simulink model "ball_impact"  (Simulink 8.1)
settings: Solver=ode4  SolverMode=SingleTasking  StartTime=0.0  StopTime=inf  FixedStep=0.0005  RelTol=1e-3
StartFcn:
  |  warndlg('Dexterit-E models cannot run under simulation. Please compile your model and run it from within Dexterit-E.');set_param(bdroot,'SimulationCommand','stop')
undefined symbols (not defined in the file or in its folder): CreateParameterTableGUI, slselsubs
libraries: xpclib x30, simulink x8, KINARM_general x3, KINARM_loads x2, Video x2, KINARM_EP_loads x1
(part 2 of 5)

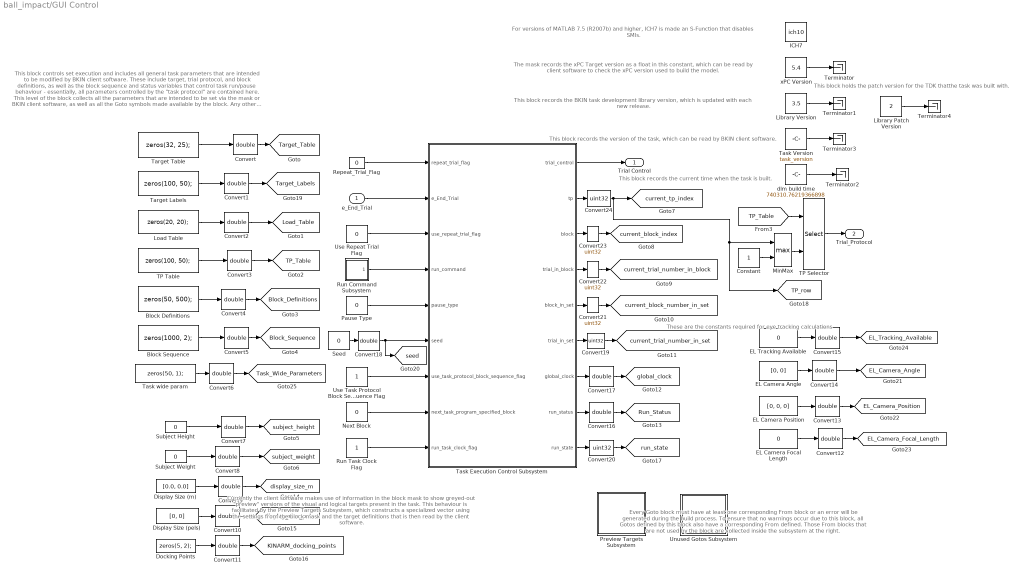
== system ball_impact/GUI Control ==
  note: This block holds the patch version for
      | the TDK thatthe task was built with.
  note: These are the constants required for eye tracking calculations
  note: This block records the version of the task,
      | which can be read by BKIN client software.
  note: This block records the BKIN task development library
      | version, which is updated with each new release.
  note: Currently the client software makes use of information in the block mask to show
      | greyed-out "preview" versions of the visual and logical targets present in the task.
      | This behaviour is facilitated by the Preview Targets Subsystem, which constructs
      | a specialized vector using the settings from the block mask and the target
      | definitions that is then read by the client software.
  note: This block controls set execution and includes all general task parameters that are intended to be modified by BKIN client software. These include
      | target, trial protocol, and block definitions, as well as the block sequence and status variables that control task run/pause behaviour - essentially, all
      | parameters controlled by the "task protocol" are contained here.
      |
      | This level of the block collects all the parameters that are intended to be set via the mask or BKIN client software, as well as all the Goto symbols
      | made available by the block. Any other parameters to be read or written outside of this block should be placed at this level. The task execution
      | control subsystem performs the actual control of task execution using these parameters.
      |
      | Those parameters used to create Goto symbols directly are collected at the left, and all other parameters are connected directly to the subsystem.
  note: The mask records the xPC Target version as a float
      | in this constant, which can be read by client software
      | to check the xPC version used to build the model.
  note: For versions of MATLAB 7.5 (R2007b) and higher,
      | ICH7 is made an S-Function that disables SMIs.
  note: Every Goto block must have at least one corresponding
      | From block or an error will be generated during the build
      | process. To ensure that no warnings occur due to this block,
      | all Gotos defined by this block also have a corresponding
      | From defined. Those From blocks that are not used by the
      | block are collected inside the subsystem at the right.
  note: This block records the current
      | time when the task is built.
  e_End_Trial : Inport
  Block Definitions : Constant  Value=zeros(50, 500);
  Block Sequence : Constant  Value=zeros(1000, 2);
  Constant : Constant  VectorParams1D=off  OutDataTypeStr=double
  Convert{,1..18} (19 alike) : DataTypeConversion  OutDataTypeStr=double
  Convert{19..24} (6 alike) : DataTypeConversion  OutDataTypeStr=uint32
  Display Size (m) : Constant  Value=[0.0, 0.0]  VectorParams1D=off  OutDataTypeStr=double
  Display Size (pels) : Constant  Value=[0, 0]  VectorParams1D=off  OutDataTypeStr=double
  Docking Points : Constant  Value=zeros(5, 2);  VectorParams1D=off  OutDataTypeStr=double
  EL Camera Angle : Constant  Value=[0, 0]  VectorParams1D=off  OutDataTypeStr=double
  EL Camera Focal Length : Constant  Value=0  VectorParams1D=off  OutDataTypeStr=double
  EL Camera Position : Constant  Value=[0, 0, 0]  VectorParams1D=off  OutDataTypeStr=double
  EL Tracking Available : Constant  Value=0  VectorParams1D=off  OutDataTypeStr=double
  ICH7 : S-Function  FunctionName=ich10  EnableBusSupport=off
  Library Patch Version : Constant  Value=2
  Library Version : Constant  Value=3.5
  Load Table : Constant  Value=zeros(20, 20);
  MinMax : MinMax  Function=max  Inputs=2
  Next Block : Constant  Value=0  VectorParams1D=off  OutDataTypeStr=double
  Pause Type : Constant  Value=0
  Preview Targets Subsystem : Subsystem
  Repeat_Trial_Flag : Constant  Value=0
  Run Command Subsystem : Subsystem
  Run Task Clock Flag : Constant  VectorParams1D=off  OutDataTypeStr=double
  Seed : Constant  Value=0
  Subject Height : Constant  Value=0  VectorParams1D=off  OutDataTypeStr=double
  Subject Weight : Constant  Value=0  VectorParams1D=off  OutDataTypeStr=double
  TP Selector : Selector  NumberOfDimensions=2  InputPortWidth=3  IndexOptions=Index vector (port),Select all  Indices=1,-1  OutputSizes=slselsubs([(-2),(-2)],1),slselsubs([(-2),(-2)],2)
  TP Table : Constant  Value=zeros(100, 50);
  Target Labels : Constant  Value=zeros(100, 50);
  Target Table : Constant  Value=zeros(32, 25);
  Task Execution Control Subsystem : Subsystem
  Task Version : Constant  Value=task_version
  Task wide param : Constant  Value=zeros(50, 1);
  Terminator{,1..4} (5 alike) : Terminator
  Unused Gotos Subsystem : Subsystem
  Use Repeat Trial Flag : Constant  Value=0
  Use Task Protocol Block Sequence Flag : Constant  VectorParams1D=off  OutDataTypeStr=double
  dlm build time : Constant  Value=740310.76219366898
  xPC Version : Constant  Value=5.4
  Trial Control : Outport
  Trial_Protocol : Outport  Port=2
  tag scope: Block_Definitions=global, Block_Sequence=global, EL_Camera_Angle=global, EL_Camera_Focal_Length=global, EL_Camera_Position=global, EL_Tracking_Available=global, KINARM_docking_points=global, Load_Table=global, Run_Status=global, TP_Table=global, TP_row=global, Target_Labels=global, Target_Table=global, Task_Wide_Parameters=global, current_block_index=global, current_block_number_in_set=global, current_tp_index=global, current_trial_number_in_block=global, current_trial_number_in_set=global, display_size_m=global, display_size_pels=global, global_clock=global, run_state=global, seed=global, subject_height=global, subject_weight=global
  wires:
  Library Patch Version/1 -> Terminator4/1
  EL Tracking Available/1 -> Convert15/1
  EL Camera Focal Length/1 -> Convert12/1
  EL Camera Position/1 -> Convert13/1
  EL Camera Angle/1 -> Convert14/1
  Task Version/1 -> Terminator3/1
  Target Labels/1 -> Convert1/1
  Task Execution Control Subsystem/9(run_state) -> Convert20/1
  Docking Points/1 -> Convert11/1
  Display Size (pels)/1 -> Convert10/1
  Display Size (m)/1 -> Convert9/1
  Constant/1 -> MinMax/2
  MinMax/1 -> TP Selector/2
  Run Task Clock Flag/1 -> Task Execution Control Subsystem/9(run_task_clock_flag)
  Use Repeat Trial Flag/1 -> Task Execution Control Subsystem/3(use_repeat_trial_flag)
  Library Version/1 -> Terminator1/1
  Subject Weight/1 -> Convert8/1
  Subject Height/1 -> Convert7/1
  Task Execution Control Subsystem/4(trial_in_block) -> Convert22/1
  Next Block/1 -> Task Execution Control Subsystem/8(next_task_program_specified_block)
  Block Sequence/1 -> Convert5/1
  TP Table/1 -> Convert3/1
  xPC Version/1 -> Terminator/1
  Target Table/1 -> Convert/1
  Block Definitions/1 -> Convert4/1
  Task Execution Control Subsystem/5(block_in_set) -> Convert21/1
  Use Task Protocol Block Sequence Flag/1 -> Task Execution Control Subsystem/7(use_task_protocol_block_sequence_flag)
  [TP_Table] -> TP Selector/1
  Task Execution Control Subsystem/6(trial_in_set) -> Convert19/1
  Task Execution Control Subsystem/3(block) -> Convert23/1
  Pause Type/1 -> Task Execution Control Subsystem/5(pause_type)
  Run Command Subsystem/1(Out1) -> Task Execution Control Subsystem/4(run_command)
  Seed/1 -> Convert18/1
  e_End_Trial/1 -> Task Execution Control Subsystem/2(e_End_Trial)
  TP Selector/1 -> Trial_Protocol/1
  Task Execution Control Subsystem/2(tp) -> Convert24/1
  Task Execution Control Subsystem/1(trial_control) -> Trial Control/1
  Load Table/1 -> Convert2/1
  Task Execution Control Subsystem/7(global_clock) -> Convert17/1
  Task Execution Control Subsystem/8(run_status) -> Convert16/1
  dlm build time/1 -> Terminator2/1
  Task wide param/1 -> Convert6/1
  Convert/1 -> [Target_Table]
  Convert1/1 -> [Target_Labels]
  Convert2/1 -> [Load_Table]
  Convert3/1 -> [TP_Table]
  Convert4/1 -> [Block_Definitions]
  Convert5/1 -> [Block_Sequence]
  Convert6/1 -> [Task_Wide_Parameters]
  Convert7/1 -> [subject_height]
  Convert8/1 -> [subject_weight]
  Convert9/1 -> [display_size_m]
  Convert10/1 -> [display_size_pels]
  Convert11/1 -> [KINARM_docking_points]
  Convert12/1 -> [EL_Camera_Focal_Length]
  Convert13/1 -> [EL_Camera_Position]
  Convert14/1 -> [EL_Camera_Angle]
  Convert15/1 -> [EL_Tracking_Available]
  Convert16/1 -> [Run_Status]
  Convert17/1 -> [global_clock]
  Convert18/1 -> [seed], Task Execution Control Subsystem/6(seed)
  Convert20/1 -> [run_state]
  Convert19/1 -> [current_trial_number_in_set]
  Convert21/1 -> [current_block_number_in_set]
  Convert22/1 -> [current_trial_number_in_block]
  Convert23/1 -> [current_block_index]
  Convert24/1 -> [TP_row], MinMax/1, [current_tp_index]
  Repeat_Trial_Flag/1 -> Task Execution Control Subsystem/1(repeat_trial_flag)

== system ball_impact/Parameter Table Defn ==
  TP_table : Subsystem
  buttons : Subsystem
  events : Subsystem
  load_table : Subsystem
  target_table : Subsystem
  task_definition : Subsystem
  task_wide : Subsystem

== system ball_impact/DataLogging/Create Analog Inputs Subsystem ==
  In1 : Inport
  Analog Data : DataTypeConversion  SaturateOnIntegerOverflow=on  RndMeth=Zero
  Analog Data Width : DataTypeConversion  SaturateOnIntegerOverflow=on  RndMeth=Zero
  Mux2 : Mux  Inputs=2
  Not Logging Analog Inputs : Constant  Value=0
  Rate Transition9 : RateTransition
  Subtract : Sum  Inputs=-+
  Width : Width
  Out1 : Outport
  wires:
  Mux2/1 -> Rate Transition9/1
  In1/1 -> Analog Data/1, Width/1
  Subtract/1 -> Analog Data Width/1
  Not Logging Analog Inputs/1 -> Subtract/1
  Analog Data Width/1 -> Mux2/1
  Width/1 -> Subtract/2
  Analog Data/1 -> Mux2/2
  Rate Transition9/1 -> Out1/1

== system ball_impact/DataLogging/Create Custom Data Subsystem ==
  In1 : Inport
  Custom Data : DataTypeConversion  SaturateOnIntegerOverflow=on  RndMeth=Zero
  Custom Data Width : DataTypeConversion  SaturateOnIntegerOverflow=on  RndMeth=Zero
  Mux6 : Mux  Inputs=2
  Rate Transition9 : RateTransition
  Width : Width
  Out1 : Outport
  wires:
  Mux6/1 -> Rate Transition9/1
  In1/1 -> Custom Data/1, Width/1
  Custom Data Width/1 -> Mux6/1
  Width/1 -> Custom Data Width/1
  Custom Data/1 -> Mux6/2
  Rate Transition9/1 -> Out1/1

== system ball_impact/DataLogging/Create Event Codes Subsystem ==
  In1 : Inport
  Event Codes : DataTypeConversion  SaturateOnIntegerOverflow=on  RndMeth=Zero
  Mux4 : Mux  Inputs=2
  Not Logging Event Codes : Constant  Value=0
  Number of Event Codes : DataTypeConversion  SaturateOnIntegerOverflow=on  RndMeth=Zero
  Rate Transition9 : RateTransition
  Subtract : Sum  Inputs=-+
  Width : Width
  Out1 : Outport
  wires:
  Mux4/1 -> Rate Transition9/1
  In1/1 -> Event Codes/1, Width/1
  Not Logging Event Codes/1 -> Subtract/1
  Subtract/1 -> Number of Event Codes/1
  Width/1 -> Subtract/2
  Number of Event Codes/1 -> Mux4/1
  Event Codes/1 -> Mux4/2
  Rate Transition9/1 -> Out1/1

== system ball_impact/DataLogging/Create KINARM Data Subsystem ==
  In1 : Inport
  Arm Kinematics : DataTypeConversion  SaturateOnIntegerOverflow=on  RndMeth=Zero
  Kinarm Data Width : DataTypeConversion  SaturateOnIntegerOverflow=on  RndMeth=Zero
  Mux : Mux  Inputs=3
  Mux1 : Mux  Inputs=2
  Mux3 : Mux
  Rate Transition4 : RateTransition
  Select Arm Data : Selector  NumberOfDimensions=2  InputPortWidth=3  IndexOptions=Index vector (dialog),Index vector (dialog)  Indices=[1, 2],[17,18,19,20,21,22,23,24,15,16, 44, 45, 46, 47, 48, 49, 50]  OutputSizes=slselsubs([(-2),(-2)],1),slselsubs([(-2),(-2)],2)
  Select Arm1 : Selector  NumberOfDimensions=2  InputPortWidth=3  IndexOptions=Index vector (dialog),Select all  Indices=1,-1  OutputSizes=slselsubs([(-2),(-2)],1),slselsubs([(-2),(-2)],2)
  Select Arm2 : Selector  NumberOfDimensions=2  InputPortWidth=3  IndexOptions=Index vector (dialog),Select all  Indices=2,-1  OutputSizes=slselsubs([(-2),(-2)],1),slselsubs([(-2),(-2)],2)
  Width : Width
  Out1 : Outport
  wires:
  Select Arm Data/1 -> Select Arm2/1, Select Arm1/1
  In1/1 -> Select Arm Data/1
  Mux1/1 -> Rate Transition4/1
  Mux3/1 -> Width/1, Arm Kinematics/1
  Select Arm2/1 -> Mux3/2
  Select Arm1/1 -> Mux3/1
  Kinarm Data Width/1 -> Mux1/1
  Width/1 -> Kinarm Data Width/1
  Arm Kinematics/1 -> Mux1/2
  [ForcePlateData] -> Mux3/4
  [Gaze_Global] -> Mux/1
  Mux/1 -> Mux3/3
  [Gaze_Event_Info] -> Mux/3
  [Gaze_pupil_area] -> Mux/2
  Rate Transition4/1 -> Out1/1

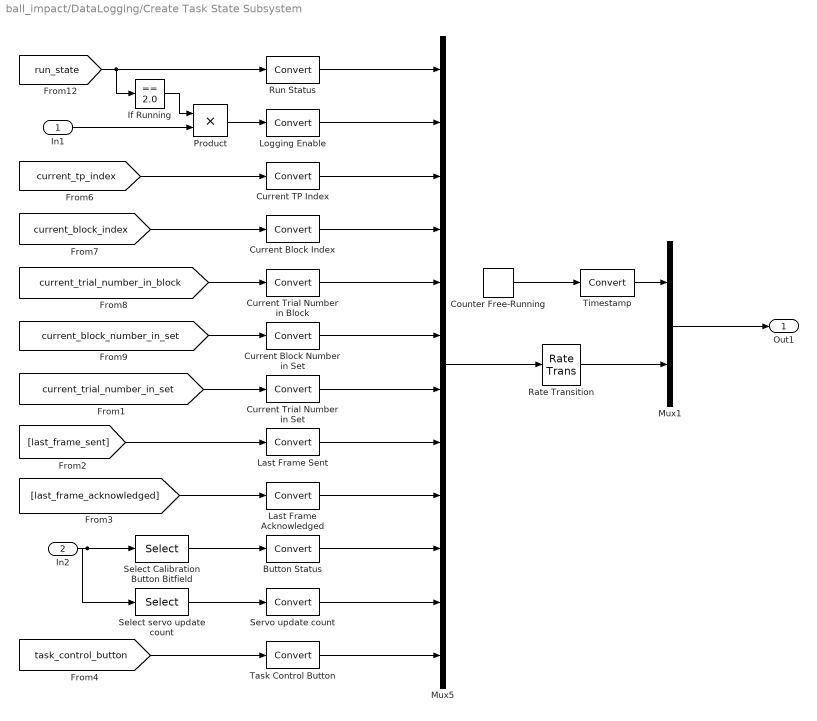
== system ball_impact/DataLogging/Create Task State Subsystem ==
  In1 : Inport
  In2 : Inport  Port=2
  Button Status : DataTypeConversion  SaturateOnIntegerOverflow=on  RndMeth=Zero
  Counter Free-Running : simulink/Sources/Counter Free-Running  NumBits=32  tsamp=-1
  Current Block Index : DataTypeConversion  SaturateOnIntegerOverflow=on  RndMeth=Zero
  Current Block Number in Set : DataTypeConversion  SaturateOnIntegerOverflow=on  RndMeth=Zero
  Current TP Index : DataTypeConversion  SaturateOnIntegerOverflow=on  RndMeth=Zero
  Current Trial Number in Block : DataTypeConversion  SaturateOnIntegerOverflow=on  RndMeth=Zero
  Current Trial Number in Set : DataTypeConversion  SaturateOnIntegerOverflow=on  RndMeth=Zero
  If Running : simulink/Logic and Bit Operations/Compare To Constant  relop===  const=2.0  OutDataTypeStr=uint8  ZeroCross=off
  Last Frame Acknowledged : DataTypeConversion  SaturateOnIntegerOverflow=on  RndMeth=Zero
  Last Frame Sent : DataTypeConversion  SaturateOnIntegerOverflow=on  RndMeth=Zero
  Logging Enable : DataTypeConversion  SaturateOnIntegerOverflow=on  RndMeth=Zero
  Mux1 : Mux  Inputs=2
  Mux5 : Mux  Inputs=12
  Product : Product  RndMeth=Zero
  Rate Transition : RateTransition
  Run Status : DataTypeConversion  SaturateOnIntegerOverflow=on  RndMeth=Zero
  Select Calibration Button Bitfield : Selector  NumberOfDimensions=2  InputPortWidth=3  IndexOptions=Index vector (dialog),Index vector (dialog)  Indices=[3],[13]  OutputSizes=slselsubs([(-2),(-2)],1),slselsubs([(-2),(-2)],2)
  Select servo update count : Selector  NumberOfDimensions=2  InputPortWidth=3  IndexOptions=Index vector (dialog),Index vector (dialog)  Indices=[3],[12]  OutputSizes=slselsubs([(-2),(-2)],1),slselsubs([(-2),(-2)],2)
  Servo update count : DataTypeConversion  SaturateOnIntegerOverflow=on  RndMeth=Zero
  Task Control Button : DataTypeConversion  SaturateOnIntegerOverflow=on  RndMeth=Zero
  Timestamp : DataTypeConversion  SaturateOnIntegerOverflow=on  RndMeth=Zero
  Out1 : Outport
  wires:
  Task Control Button/1 -> Mux5/12
  [task_control_button] -> Task Control Button/1
  In2/1 -> Select Calibration Button Bitfield/1, Select servo update count/1
  Button Status/1 -> Mux5/10
  Select Calibration Button Bitfield/1 -> Button Status/1
  [last_frame_acknowledged] -> Last Frame Acknowledged/1
  [last_frame_sent] -> Last Frame Sent/1
  Last Frame Acknowledged/1 -> Mux5/9
  Last Frame Sent/1 -> Mux5/8
  In1/1 -> Product/2
  Current Trial Number in Set/1 -> Mux5/7
  Current Block Number in Set/1 -> Mux5/6
  Current Trial Number in Block/1 -> Mux5/5
  Current Block Index/1 -> Mux5/4
  Current TP Index/1 -> Mux5/3
  Logging Enable/1 -> Mux5/2
  Run Status/1 -> Mux5/1
  [current_trial_number_in_set] -> Current Trial Number in Set/1
  [current_block_number_in_set] -> Current Block Number in Set/1
  [current_trial_number_in_block] -> Current Trial Number in Block/1
  [current_block_index] -> Current Block Index/1
  [current_tp_index] -> Current TP Index/1
  If Running/1 -> Product/1
  Counter Free-Running/1 -> Timestamp/1
  [run_state] -> If Running/1, Run Status/1
  Product/1 -> Logging Enable/1
  Servo update count/1 -> Mux5/11
  Select servo update count/1 -> Servo update count/1
  Mux1/1 -> Out1/1
  Timestamp/1 -> Mux1/1
  Mux5/1 -> Rate Transition/1
  Rate Transition/1 -> Mux1/2

== system ball_impact/DataLogging/Keep alive ==
  note: Every 100ms this sends out a message that
      | DexDisplay should get and replay to Dex.
      | That is how Dex can tell if DexDisplay is blocked by a firewall.
  Pack : xpclib/UDP/Pack  datatypes={'double'}  byteAlign=1
  Send : xpclib/UDP/Send  ipAddress=192.168.0.1  ipPort=50010  localPort=-1  vblLen=off  sampletime=0.1
  const : Constant  Value=[1 1 1 1 1]  OutDataTypeStr=double
  wires:
  const/1 -> Pack/1
  Pack/1 -> Send/1

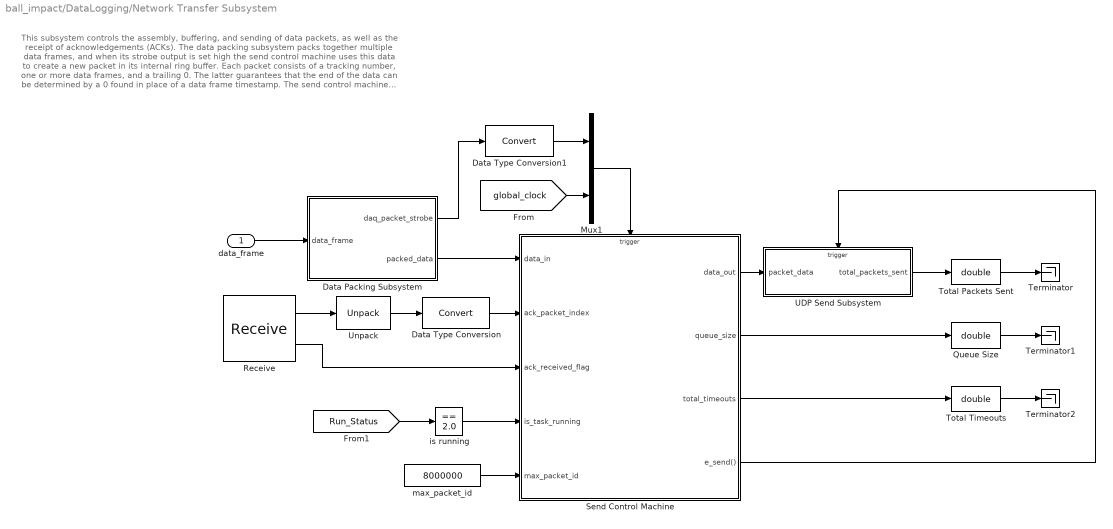
== system ball_impact/DataLogging/Network Transfer Subsystem ==
  note: This subsystem controls the assembly, buffering, and sending of data packets, as well as the receipt of acknowledgements (ACKs). The data packing subsystem packs
      | together multiple data frames, and when its strobe output is set high the send control machine uses this data to create a new packet in its internal ring buffer. Each
      | packet consists of a tracking number, one or more data frames, and a trailing 0. The latter guarantees that the end of the data can be determined by a 0 found in
      | place of a data frame timestamp.
      |
      | The send control machine will send the next packet in its buffer after an ACK for the previous one is received. If it  will resend a packet if it has not received an ACK
      | after a fixed time, and repeat the send for every elapse of that time. Currently up to 5000 packets - a minimum of 5 seconds and a maximum of 30 seconds of data,
      | depending on frame size - are buffered.
  data_frame : Inport
  Data Packing Subsystem : Subsystem  TreatAsAtomicUnit=on  SystemSampleTime=0.001
  Data Type Conversion : DataTypeConversion
  Data Type Conversion1 : DataTypeConversion
  Mux1 : Mux  Inputs=2
  Queue Size : DataTypeConversion  OutDataTypeStr=double  SaturateOnIntegerOverflow=on  RndMeth=Zero
  Receive : xpclib/UDP/Receive  ipAddress=192.168.0.1  ipPort=50001  width=4  vblLen=off  sampletime=BKIN_STEP_TIME
  Send Control Machine : Stateflow chart  TreatAsAtomicUnit=on
  Terminator : Terminator
  Terminator1 : Terminator
  Terminator2 : Terminator
  Total Packets Sent : DataTypeConversion  OutDataTypeStr=double  SaturateOnIntegerOverflow=on  RndMeth=Zero
  Total Timeouts : DataTypeConversion  OutDataTypeStr=double  SaturateOnIntegerOverflow=on  RndMeth=Zero
  UDP Send Subsystem : Subsystem  TreatAsAtomicUnit=on
  Unpack : xpclib/UDP/Unpack  dimensions={[1]}  datatypes={'single'}  byteAlign=1
  is running : simulink/Logic and Bit Operations/Compare To Constant  relop===  const=2.0  OutDataTypeStr=uint8  ZeroCross=off
  max_packet_id : Constant  Value=8000000  OutDataTypeStr=uint32
  wires:
  is running/1 -> Send Control Machine/4(is_task_running)
  [Run_Status] -> is running/1
  Data Type Conversion1/1 -> Mux1/1
  Total Packets Sent/1 -> Terminator/1
  Queue Size/1 -> Terminator1/1
  Data Type Conversion/1 -> Send Control Machine/2(ack_packet_index)
  Receive/2 -> Send Control Machine/3(ack_received_flag)
  Send Control Machine/1(data_out) -> UDP Send Subsystem/1(packet_data)
  Send Control Machine/4(e_send()) -> UDP Send Subsystem/Trigger
  Data Packing Subsystem/1(daq_packet_strobe) -> Data Type Conversion1/1
  [global_clock] -> Mux1/2
  Send Control Machine/2(queue_size) -> Queue Size/1
  Send Control Machine/3(total_timeouts) -> Total Timeouts/1
  Mux1/1 -> Send Control Machine/Trigger
  Receive/1 -> Unpack/1
  Unpack/1 -> Data Type Conversion/1
  Data Packing Subsystem/2(packed_data) -> Send Control Machine/1(data_in)
  data_frame/1 -> Data Packing Subsystem/1(data_frame)
  UDP Send Subsystem/1(total_packets_sent) -> Total Packets Sent/1
  Total Timeouts/1 -> Terminator2/1
  max_packet_id/1 -> Send Control Machine/5(max_packet_id)

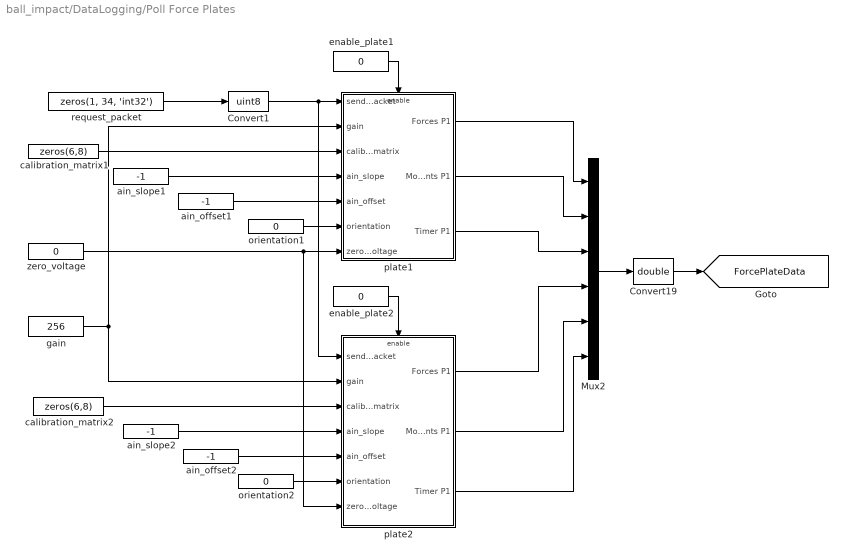
== system ball_impact/DataLogging/Poll Force Plates ==
  Convert1 : DataTypeConversion  OutDataTypeStr=uint8
  Convert19 : DataTypeConversion  OutDataTypeStr=double
  Mux2 : Mux  Inputs=6
  ain_offset1 : Constant  Value=-1
  ain_offset2 : Constant  Value=-1
  ain_slope1 : Constant  Value=-1
  ain_slope2 : Constant  Value=-1
  calibration_matrix1 : Constant  Value=zeros(6,8)
  calibration_matrix2 : Constant  Value=zeros(6,8)
  enable_plate1 : Constant  Value=0
  enable_plate2 : Constant  Value=0
  gain : Constant  Value=256
  orientation1 : Constant  Value=0
  orientation2 : Constant  Value=0
  plate1 : Subsystem
  plate2 : Subsystem
  request_packet : Constant  Value=zeros(1, 34, 'int32')
  zero_voltage : Constant  Value=0
  tag scope: ForcePlateData=global
  wires:
  gain/1 -> plate2/2(gain), plate1/2(gain)
  plate1/1(Forces P1) -> Mux2/1
  plate1/2(Moments P1) -> Mux2/2
  plate1/3(Timer P1) -> Mux2/3
  plate2/1(Forces P1) -> Mux2/4
  plate2/2(Moments P1) -> Mux2/5
  plate2/3(Timer P1) -> Mux2/6
  calibration_matrix1/1 -> plate1/3(calib_matrix)
  calibration_matrix2/1 -> plate2/3(calib_matrix)
  enable_plate1/1 -> plate1/Enable
  enable_plate2/1 -> plate2/Enable
  Mux2/1 -> Convert19/1
  ain_slope1/1 -> plate1/4(ain_slope)
  ain_offset1/1 -> plate1/5(ain_offset)
  ain_slope2/1 -> plate2/4(ain_slope)
  ain_offset2/1 -> plate2/5(ain_offset)
  orientation1/1 -> plate1/6(orientation)
  orientation2/1 -> plate2/6(orientation)
  Convert19/1 -> [ForcePlateData]
  Convert1/1 -> plate1/1(send_packet), plate2/1(send_packet)
  request_packet/1 -> Convert1/1
  zero_voltage/1 -> plate1/7(zero_voltage), plate2/7(zero_voltage)

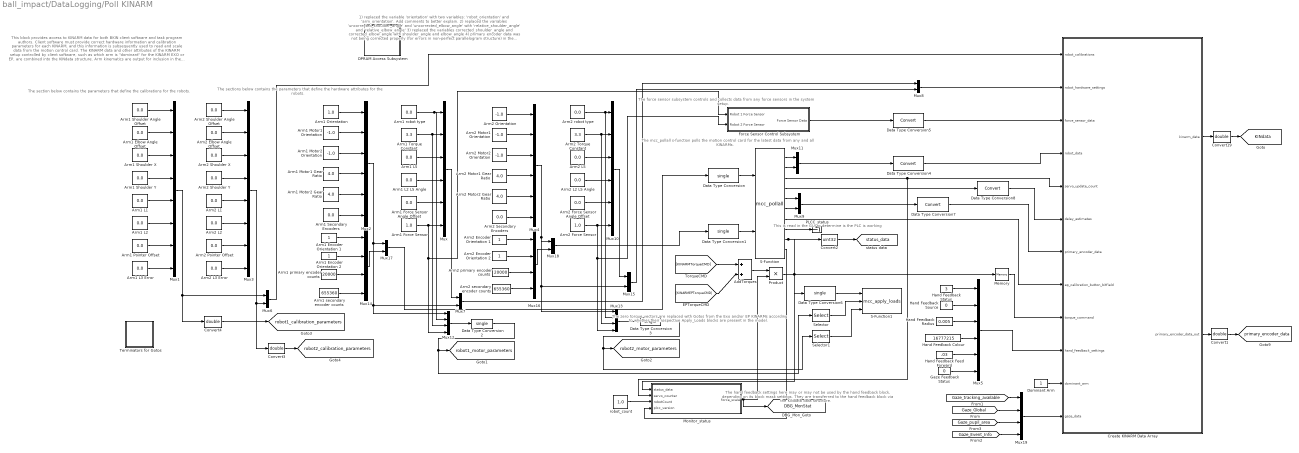
== system ball_impact/DataLogging/Poll KINARM ==
  note: This block provides access to KINARM data for both BKIN client software and task program authors. Client software must provide
      | correct hardware information and calibration parameters for each KINARM, and this information is subsequently used to read
      | and scale data from the motion control card. The KINARM data and other attributes of the KINARM setup controlled by client
      | software, such as which arm is "dominant" for the KINARM EXO or EP, are combined into the KINdata structure. Arm kinematics
      | are output for inclusion in the current data frame.
      |
      | This block also offers client software access to the motion control card DPRAM via the DPRAM access subsystem.
      |
      | Note: The mask replaces the ZeroTorque constant with a From block that includes the commanded torques providing the model
      | includes an instance of the load-applying block.
      |
      | Note: For each Goto block created here, a corresponding From block is included in the Terminators for Gotos subsystem. This is
      | solely to prevent unnecessary warnings at the Matlab prompt if such From blocks are not present.
  note: The mcc_pollall s-function polls the motion control
      | card for the latest data from any and all KINARMs.
  note: The section below contains the parameters that define the calibrations for the robots.
  note: The sections below contains the parameters that define the hardware attributes for the robots.
  note: The hand feedback settings here may or may not be used by the hand
      | feedback block, depending on its block mask settings. They are
      | transferred to the hand feedback block via the KINdata data structure.
  note: The force sensor subsystem controls and collects
      | data from any force sensors in the system setup.
  note: The zero torque vectors are replaced with Gotos
      | from the Exo and/or EP KINARMs according to
      | whether their respective Apply_Loads blocks are
      | present in the model.
  note: 1) replaced the variable 'orientation' with two variables: 'robot_orientation' and 'arm_orientation'.  Add comments to better explain.
      | 2) replaced the variables 'uncorrected_shoulder_angle' and 'uncorrected_elbow_angle' with 'relative_shoulder_angle' and 'relative_elbow_angle'
      | 3) replaced the variables corrected_shoulder_angle and corrected_elbow_angle with shoulder_angle and elbow_angle
      | 4) primary encoder data was not being corrected properly (for errors in non-perfect parallelogram structure) in the original.  This has now been fixed.
      | 5) replaced "if (robot_type < 1.0 && orientation == 2) || (robot_type > 0.0 && orientation == 1)"
      |             with "(robot_orientation == -1)"
  note: This is read in the GUI to determine is the PLC is working
  AddTorques : Sum
  Arm1 Elbow Angle Offset : Constant  Value=0.0
  Arm1 Encoder Orientation 1 : Constant
  Arm1 Encoder Orientation 2 : Constant
  Arm1 Force Sensor : Constant  Value=1.0
  Arm1 Force Sensor Angle Offset : Constant  Value=0.0
  Arm1 L1 : Constant  Value=0.0
  Arm1 L2 : Constant  Value=0.0
  Arm1 L2 L5 Angle : Constant  Value=0.0
  Arm1 L3 Error : Constant  Value=0.0
  Arm1 L5 : Constant  Value=0.0
  Arm1 Motor1 Gear Ratio : Constant  Value=4.0
  Arm1 Motor1 Orientation : Constant  Value=-1.0
  Arm1 Motor2 Gear Ratio : Constant  Value=4.0
  Arm1 Motor2 Orientation : Constant  Value=-1.0
  Arm1 Orientation : Constant  Value=1.0
  Arm1 Pointer Offset : Constant  Value=0.0
  Arm1 Secondary Encoders : Constant  Value=0.0
  Arm1 Shoulder Angle Offset : Constant  Value=0.0
  Arm1 Shoulder X : Constant  Value=0.0
  Arm1 Shoulder Y : Constant  Value=0.0
  Arm1 Torque Constant : Constant  Value=3.3
  Arm1 primary encoder counts : Constant  Value=20000
  Arm1 robot type : Constant  Value=0.0
  Arm1 secondary encoder counts : Constant  Value=655360
  Arm2 Elbow Angle Offset : Constant  Value=0.0
  Arm2 Encoder Orientation 1 : Constant
  Arm2 Encoder Orientation 2 : Constant
  Arm2 Force Sensor : Constant  Value=1.0
  Arm2 Force Sensor Angle Offset : Constant  Value=0.0
  Arm2 L1 : Constant  Value=0.0
  Arm2 L2 : Constant  Value=0.0
  Arm2 L2 L5 Angle : Constant  Value=0.0
  Arm2 L3 Error : Constant  Value=0.0
  Arm2 L5 : Constant  Value=0.0
  Arm2 Motor1 Gear Ratio : Constant  Value=4.0
  Arm2 Motor1 Orientation : Constant  Value=-1.0
  Arm2 Motor2 Gear Ratio : Constant  Value=4.0
  Arm2 Motor2 Orientation : Constant  Value=-1.0
  Arm2 Orientation : Constant  Value=-1.0
  Arm2 Pointer Offset : Constant  Value=0.0
  Arm2 Secondary Encoders : Constant  Value=0.0
  Arm2 Shoulder Angle Offset : Constant  Value=0.0
  Arm2 Shoulder X : Constant  Value=0.0
  Arm2 Shoulder Y : Constant  Value=0.0
  Arm2 Torque Constant : Constant  Value=3.3
  Arm2 primary encoder counts : Constant  Value=20000
  Arm2 robot type : Constant  Value=0.0
  Arm2 secondary encoder counts : Constant  Value=655360
  Convert{1,3..4,19} (4 alike) : DataTypeConversion  OutDataTypeStr=double
  Convert2 : DataTypeConversion  OutDataTypeStr=uint32
  Create KINARM Data Array : MATLAB Function  TreatAsAtomicUnit=on
  DPRAM Access Subsystem : Subsystem
  Data Type Conversion{,1..3,6} (5 alike) : DataTypeConversion  OutDataTypeStr=single
  Data Type Conversion{4..5,7..8} (4 alike) : DataTypeConversion
  Dominant Arm : Constant
  Force Sensor Control Subsystem : Subsystem
  Gaze Feedback Status : Constant  Value=0
  Hand Feedback Colour : Constant  Value=16777215
  Hand Feedback Feed Forward : Constant  Value=.03
  Hand Feedback Radius : Constant  Value=0.005
  Hand Feedback Source : Constant  Value=0
  Hand Feedback Status : Constant  Value=3
  Memory : Memory
  Monitor_status : MATLAB Function  TreatAsAtomicUnit=on  SystemSampleTime=.001
  Mux{,2,4..5,10} (5 alike) : Mux  Inputs=6
  Mux1 : Mux  Inputs=8
  Mux{6..9,11,15,17..18} (8 alike) : Mux  Inputs=2
  Mux{12..14,16,19} (5 alike) : Mux
  Mux3 : Mux  Inputs=8
  PLCC_status : Terminator
  Product : Product  RndMeth=Zero
  S-Function : S-Function  FunctionName=mcc_pollall  EnableBusSupport=off
  S-Function1 : S-Function  FunctionName=mcc_apply_loads  EnableBusSupport=off
  Selector : Selector  InputPortWidth=9  IndexOptions=Index vector (dialog)  Indices=[1, 2, 3, 4, 5, 8]  OutputSizes=[(-2)]
  Selector1 : Selector  InputPortWidth=9  IndexOptions=Index vector (dialog)  Indices=[1, 2, 3, 4, 5, 8]  OutputSizes=[(-2)]
  Terminators for Gotos : Subsystem
  robot_count : Constant  Value=1.0
  tag scope: DBG_MonStat=global, KINdata=global, primary_encoder_data=global, robot1_calibration_parameters=global, robot1_motor_parameters=global, robot2_calibration_parameters=global, robot2_motor_parameters=global, status_data=global
  wires:
  Arm2 secondary encoder counts/1 -> Mux16/4
  Arm2 primary encoder counts/1 -> Mux16/3
  Arm1 secondary encoder counts/1 -> Mux14/4
  Arm1 primary encoder counts/1 -> Mux14/3
  Arm1 Shoulder Angle Offset/1 -> Mux1/1
  Arm1 Elbow Angle Offset/1 -> Mux1/2
  Arm1 Shoulder X/1 -> Mux1/3
  Arm1 Shoulder Y/1 -> Mux1/4
  Arm1 L1/1 -> Mux1/5
  Arm1 L2/1 -> Mux1/6
  Arm1 Pointer Offset/1 -> Mux1/7
  Arm1 L3 Error/1 -> Mux1/8
  Arm2 Shoulder Angle Offset/1 -> Mux3/1
  Arm2 Elbow Angle Offset/1 -> Mux3/2
  Arm2 Shoulder X/1 -> Mux3/3
  Arm2 Shoulder Y/1 -> Mux3/4
  Arm2 L1/1 -> Mux3/5
  Arm2 L2/1 -> Mux3/6
  Arm2 Pointer Offset/1 -> Mux3/7
  Arm2 L3 Error/1 -> Mux3/8
  Hand Feedback Status/1 -> Mux5/1
  Hand Feedback Source/1 -> Mux5/2
  Hand Feedback Radius/1 -> Mux5/3
  Hand Feedback Colour/1 -> Mux5/4
  Hand Feedback Feed Forward/1 -> Mux5/5
  Create KINARM Data Array/1(kinarm_data) -> Convert19/1
  Arm1 Orientation/1 -> Mux2/1
  Arm1 Motor1 Orientation/1 -> Mux2/2
  Arm1 Motor2 Orientation/1 -> Mux2/3
  Arm1 Motor1 Gear Ratio/1 -> Mux2/4
  Arm1 Motor2 Gear Ratio/1 -> Mux2/5
  Arm1 Secondary Encoders/1 -> Mux2/6
  Arm2 Orientation/1 -> Mux4/1
  Arm2 Motor1 Orientation/1 -> Mux4/2
  Arm2 Motor2 Orientation/1 -> Mux4/3
  Arm2 Motor1 Gear Ratio/1 -> Mux4/4
  Arm2 Motor2 Gear Ratio/1 -> Mux4/5
  Arm2 Secondary Encoders/1 -> Mux4/6
  Arm1 robot type/1 -> Mux/1, Mux12/2
  Arm1 Torque Constant/1 -> Mux/2, Mux12/3
  Arm1 L5/1 -> Mux/3
  Arm1 L2 L5 Angle/1 -> Mux/4
  Arm2 robot type/1 -> Mux10/1, Mux13/2
  Arm2 Torque Constant/1 -> Mux10/2, Mux13/3
  Arm2 L5/1 -> Mux10/3
  Arm2 L2 L5 Angle/1 -> Mux10/4
  Arm2 Force Sensor/1 -> Mux10/6, Force Sensor Control Subsystem/2(Robot 2 Force Sensor), Mux13/4
  Dominant Arm/1 -> Create KINARM Data Array/11(dominant_arm)
  Memory/1 -> Create KINARM Data Array/9(torque_command)
  Mux5/1 -> Create KINARM Data Array/10(hand_feedback_settings)
  Mux/1 -> Mux7/1
  Mux2/1 -> Mux17/1, Mux12/1, Mux7/2
  Mux10/1 -> Mux15/1
  Mux4/1 -> Mux18/1, Mux13/1, Mux15/2
  Mux11/1 -> Data Type Conversion4/1
  Force Sensor Control Subsystem/1(Force Sensor Data) -> Data Type Conversion5/1
  Arm1 Force Sensor/1 -> Mux/6, Force Sensor Control Subsystem/1(Robot 1 Force Sensor), Mux12/4
  Arm1 Force Sensor Angle Offset/1 -> Mux/5
  Arm2 Force Sensor Angle Offset/1 -> Mux10/5
  Mux7/1 -> Mux8/1
  Mux15/1 -> Mux8/2
  Mux8/1 -> Create KINARM Data Array/2(robot_hardware_settings)
  S-Function/1 -> Mux11/1
  S-Function/2 -> Mux11/2
  S-Function/3 -> Create KINARM Data Array/5(servo_update_count), Monitor_status/2(servo_counter)
  S-Function/4 -> Data Type Conversion8/1
  Data Type Conversion1/1 -> S-Function/2
  Mux9/1 -> Data Type Conversion7/1
  Mux1/1 -> Mux6/1, Convert4/1
  Mux3/1 -> Mux6/2, Convert3/1
  Mux6/1 -> Create KINARM Data Array/1(robot_calibrations)
  Data Type Conversion/1 -> S-Function/1
  Mux12/1 -> Data Type Conversion2/1
  Data Type Conversion2/1 -> [robot1_motor_parameters], Selector/1
  Mux13/1 -> Data Type Conversion3/1
  Data Type Conversion3/1 -> [robot2_motor_parameters], Selector1/1
  S-Function/5 -> Mux9/1
  S-Function/6 -> Mux9/2
  S-Function/7 -> Create KINARM Data Array/8(ep_calibration_button_bitfield)
  Data Type Conversion4/1 -> Create KINARM Data Array/4(robot_data)
  Data Type Conversion5/1 -> Create KINARM Data Array/3(force_sensor_data)
  Create KINARM Data Array/2(primary_encoder_data_out) -> Convert1/1
  Selector1/1 -> S-Function1/3
  Selector/1 -> S-Function1/2
  Data Type Conversion6/1 -> S-Function1/1
  Arm1 Encoder Orientation 1/1 -> Mux14/1
  Arm1 Encoder Orientation 2/1 -> Mux14/2
  Arm2 Encoder Orientation 1/1 -> Mux16/1
  Arm2 Encoder Orientation 2/1 -> Mux16/2
  Mux14/1 -> Mux17/2
  Mux17/1 -> Data Type Conversion/1
  Mux16/1 -> Mux18/2
  Mux18/1 -> Data Type Conversion1/1
  Gaze Feedback Status/1 -> Mux5/6
  Data Type Conversion7/1 -> Create KINARM Data Array/7(primary_encoder_data)
  Data Type Conversion8/1 -> Create KINARM Data Array/6(delay_estimates)
  AddTorques/1 -> Product/1
  Monitor_status/1(force_scale) -> Product/2, [DBG_MonStat]
  Product/1 -> Memory/1, Data Type Conversion6/1
  S-Function/9 -> Monitor_status/1(status_data), Convert2/1
  S-Function/8 -> PLCC_status/1
  robot_count/1 -> Monitor_status/3(robotCount)
  S-Function/10 -> Monitor_status/4(plcc_version)
  [Gaze_tracking_available] -> Mux19/1
  [Gaze_Global] -> Mux19/2
  [Gaze_Event_Info] -> Mux19/4
  [Gaze_pupil_area] -> Mux19/3
  Mux19/1 -> Create KINARM Data Array/12(gaze_data)
  Convert19/1 -> [KINdata]
  Convert1/1 -> [primary_encoder_data]
  Convert2/1 -> [status_data]
  Convert3/1 -> [robot2_calibration_parameters]
  Convert4/1 -> [robot1_calibration_parameters]
  [KINARMTorqueCMD] -> AddTorques/1
  [KINARMEPTorqueCMD] -> AddTorques/2

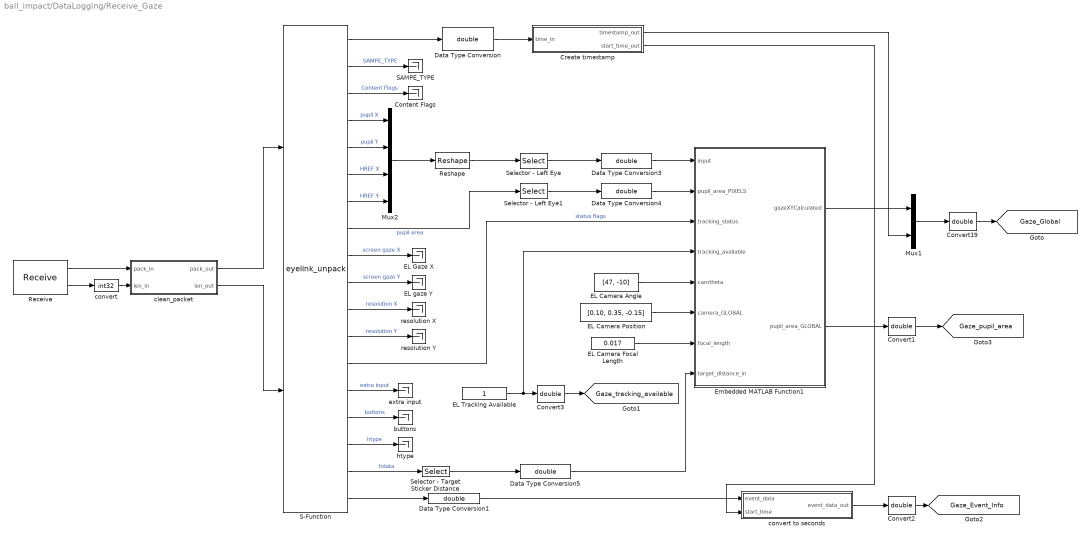
== system ball_impact/DataLogging/Receive_Gaze ==
  Content Flags : Terminator
  Convert{1..3,19} (4 alike) : DataTypeConversion  OutDataTypeStr=double
  Create timestamp : MATLAB Function  TreatAsAtomicUnit=on
  Data Type Conversion{,1,3..5} (5 alike) : DataTypeConversion  OutDataTypeStr=double
  EL Camera Angle : Constant  Value=[47, -10]  VectorParams1D=off  OutDataTypeStr=double
  EL Camera Focal Length : Constant  Value=0.017  VectorParams1D=off  OutDataTypeStr=double
  EL Camera Position : Constant  Value=[0.10, 0.35, -0.15]  VectorParams1D=off  OutDataTypeStr=double
  EL Gaze X : Terminator
  EL Tracking Available : Constant  VectorParams1D=off  OutDataTypeStr=double
  EL gaze Y : Terminator
  Embedded MATLAB Function1 : MATLAB Function  TreatAsAtomicUnit=on
  Mux1 : Mux  Inputs=2
  Mux2 : Mux
  Receive : xpclib/UDP/Receive  ipAddress=0.0.0.0  ipPort=4000  width=512  vblLen=on  sampletime=BKIN_STEP_TIME
  Reshape : Reshape  OutputDimensionality=Customize  OutputDimensions=[2,4]
  S-Function : S-Function  FunctionName=eyelink_unpack  EnableBusSupport=off
  SAMPE_TYPE : Terminator
  Selector - Left Eye : Selector  NumberOfDimensions=2  InputPortWidth=3  IndexOptions=Index vector (dialog),Index vector (dialog)  Indices=1,-1  OutputSizes=1,1
  Selector - Left Eye1 : Selector  IndexOptions=Index vector (dialog)  Indices=1  OutputSizes=1
  Selector - Target Sticker Distance : Selector  IndexOptions=Index vector (dialog)  Indices=3  OutputSizes=1
  buttons : Terminator
  clean_packet : MATLAB Function  TreatAsAtomicUnit=on
  convert : DataTypeConversion  OutDataTypeStr=int32
  convert to seconds : MATLAB Function  TreatAsAtomicUnit=on
  extra input : Terminator
  htype : Terminator
  resolution X : Terminator
  resolution Y : Terminator
  tag scope: Gaze_Event_Info=global, Gaze_Global=global, Gaze_pupil_area=global, Gaze_tracking_available=global
  wires:
  EL Tracking Available/1 -> Embedded MATLAB Function1/4(tracking_available), Convert3/1
  EL Camera Position/1 -> Embedded MATLAB Function1/6(camera_GLOBAL)
  EL Camera Angle/1 -> Embedded MATLAB Function1/5(camtheta)
  Selector - Target Sticker Distance/1 -> Data Type Conversion5/1
  Selector - Left Eye/1 -> Data Type Conversion3/1
  Reshape/1 -> Selector - Left Eye/1
  Mux2/1 -> Reshape/1
  S-Function/7 -> Mux2/4  "HREF Y"
  S-Function/6 -> Mux2/3  "HREF X"
  S-Function/5 -> Mux2/2  "pupil Y"
  S-Function/4 -> Mux2/1  "pupil X"
  Receive/2 -> convert/1
  S-Function/17 -> Selector - Target Sticker Distance/1  "hdata"
  S-Function/16 -> htype/1  "htype"
  S-Function/15 -> buttons/1  "buttons"
  S-Function/14 -> extra input/1  "extra input"
  S-Function/13 -> Embedded MATLAB Function1/3(tracking_status)  "status flags"
  S-Function/12 -> resolution Y/1  "resolution Y"
  S-Function/11 -> resolution X/1  "resolution X"
  S-Function/8 -> Selector - Left Eye1/1  "pupil area"
  S-Function/3 -> Content Flags/1  "Content Flags"
  S-Function/2 -> SAMPE_TYPE/1  "SAMPE_TYPE"
  S-Function/9 -> EL Gaze X/1  "screen gaze X"
  S-Function/10 -> EL gaze Y/1  "screen gaze Y"
  Mux1/1 -> Convert19/1
  Embedded MATLAB Function1/1(gazeXYCalculated) -> Mux1/1
  Create timestamp/1(timestamp_out) -> Mux1/2
  Data Type Conversion/1 -> Create timestamp/1(time_in)
  S-Function/1 -> Data Type Conversion/1
  S-Function/18 -> Data Type Conversion1/1
  Data Type Conversion1/1 -> convert to seconds/1(event_data)
  convert to seconds/1(event_data_out) -> Convert2/1
  Create timestamp/2(start_time_out) -> convert to seconds/2(start_time)
  Data Type Conversion3/1 -> Embedded MATLAB Function1/1(input)
  Data Type Conversion5/1 -> Embedded MATLAB Function1/8(target_distance_in)
  Embedded MATLAB Function1/2(pupil_area_GLOBAL) -> Convert1/1
  Data Type Conversion4/1 -> Embedded MATLAB Function1/2(pupil_area_PIXELS)
  EL Camera Focal Length/1 -> Embedded MATLAB Function1/7(focal_length)
  Selector - Left Eye1/1 -> Data Type Conversion4/1
  Receive/1 -> clean_packet/1(pack_in)
  convert/1 -> clean_packet/2(len_in)
  clean_packet/1(pack_out) -> S-Function/1
  clean_packet/2(len_out) -> S-Function/2
  Convert19/1 -> [Gaze_Global]
  Convert1/1 -> [Gaze_pupil_area]
  Convert2/1 -> [Gaze_Event_Info]
  Convert3/1 -> [Gaze_tracking_available]

== system ball_impact/GUI Control/Preview Targets Subsystem ==
  note: This subsystem produces a vector that defines "preview" versions of the visual and logical targets that will be used during the task.
      | This vector includes all the information needed to draw the targets, taken from the target table according to the way attributes are
      | defined for the selected target type in the mask. It is intended to be read directly by client software using the xPC API.
  Concatenation : Concatenate  Mode=Multidimensional array
  Concatenation1 : Concatenate  Mode=Multidimensional array  ConcatenateDimension=2
  Create Target Vector : MATLAB Function  TreatAsAtomicUnit=on
  L_cols : Constant  Value=Lcols
  Reshape : Reshape  OutputDimensionality=Row vector (2-D)
  Reshape1 : Reshape  OutputDimensionality=Row vector (2-D)
  Target_Type : Constant  Value=Target_Type
  Terminator : Terminator
  Terminator1 : Terminator
  V_cols : Constant  Value=Vcols
  XY_cols : Constant  Value=XYcols
  indices_padding : Constant  Value=indices_padding
  wires:
  Create Target Vector/2(target_vector_length) -> Terminator1/1
  Create Target Vector/1(target_vector) -> Terminator/1
  Concatenation1/1 -> Create Target Vector/4(attrib_column_indices)
  [Target_Table] -> Create Target Vector/1(target_table)
  Reshape/1 -> Concatenation/2
  L_cols/1 -> Reshape/1
  Reshape1/1 -> Concatenation/1
  V_cols/1 -> Reshape1/1
  Concatenation/1 -> Concatenation1/1
  indices_padding/1 -> Concatenation1/2
  XY_cols/1 -> Create Target Vector/3(xy_column_indices)
  Target_Type/1 -> Create Target Vector/2(target_type)

== system ball_impact/GUI Control/Run Command Subsystem ==
  note: This UDP receive must run at 1Khz so that
      | received signals are high for one cycle in Stateflow
  Data Type Conversion : DataTypeConversion  OutDataTypeStr=double
  Data Type Conversion1 : DataTypeConversion  OutDataTypeStr=uint8
  Data Type Conversion2 : DataTypeConversion  OutDataTypeStr=double
  Embedded MATLAB Function : MATLAB Function  TreatAsAtomicUnit=on
  Rate Transition : RateTransition  OutPortSampleTime=BKIN_STEP_TIME
  Run Command Receive : xpclib/UDP/Receive  ipAddress=0.0.0.0  ipPort=50003  width=1  vblLen=off  sampletime=0.001
  Terminator2 : Terminator
  Out1 : Outport
  tag scope: task_control_button=global
  wires:
  Data Type Conversion2/1 -> [task_control_button]
  Data Type Conversion1/1 -> Out1/1
  Data Type Conversion/1 -> Embedded MATLAB Function/1(x)
  Embedded MATLAB Function/2(z) -> Data Type Conversion2/1
  Embedded MATLAB Function/1(y) -> Data Type Conversion1/1
  Run Command Receive/1 -> Rate Transition/1
  Run Command Receive/2 -> Terminator2/1
  Rate Transition/1 -> Data Type Conversion/1

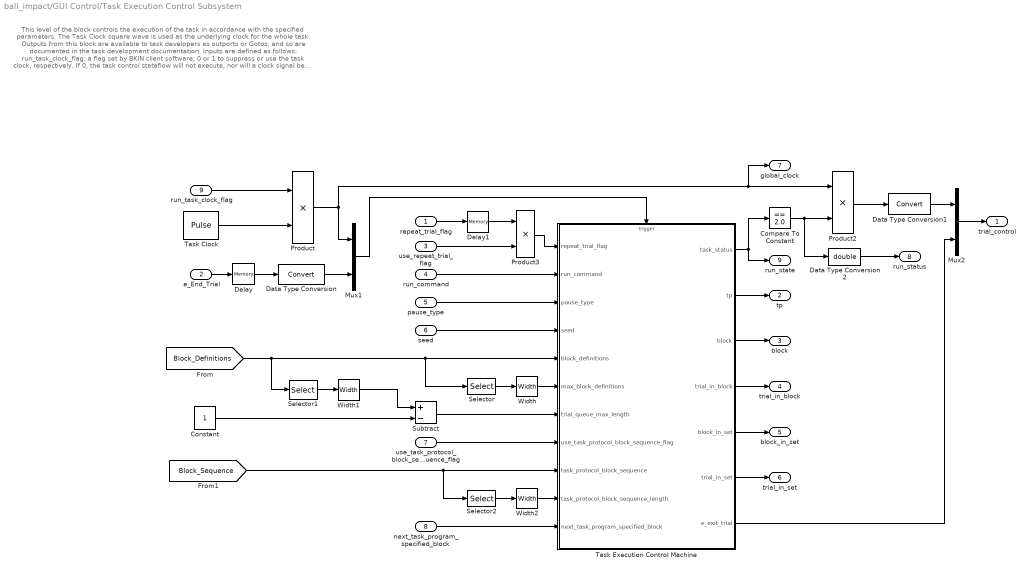
== system ball_impact/GUI Control/Task Execution Control Subsystem ==
  note: This level of the block controls the execution of the task in accordance with the specified parameters. The Task Clock square wave is used as the underlying clock for the whole task. Outputs from this block are available to task developers as
      | outports or Gotos, and so are documented in the task development documentation. Inputs are defined as follows:
      |
      | run_task_clock_flag: a flag set by BKIN client software; 0 or 1 to suppress or use the task clock, respectively. If 0, the task control stateflow will not execute, nor will a clock signal be generated for this block's trial control output or the global_clock
      | output. A setting of 0 will also stop other library blocks from sending information out via UDP.
      |
      | e_end_Trial: an user-input event that causes the control machine to, if in a trial, leave that trial and advance to the next.
      |
      | repeat_trial_flag: a user-input flag that is used when the e_end_Trial event is observed. If 1 at that time, the current TP will be added to a list of TPs that will be executed at the end of the block; if 0, no addition will happen. These repeat TPs
      | are part of the same block, but are treated together as a group once the original block completes. They are either randomized all together or not at all according to the original block's definition. Repeat TPs may be added indefinitely.
      |
      | use_repeat_trial_flag: a flag set by BKIN client software; 0 or 1 to override (suppress) repeat trials or allow them, respectively. This setting is part of task protocols.
      |
      | run_command: a value sent by BKIN client software; 0 or 1 to pause or run the task, respectively. This flag is used to run or pause the task in response to the input of users. The flag run_task_clock_flag, in contrast, is used to stop and start execution of all
      | library blocks without stopping and starting the entire model (thus losing its state).
      |
      | pause_type: an integer value in [0,4] set by BKIN client software to specify what action to take when run_flag is changed from 1 to 0 during a set. This setting is part of task protocols.
      |
      | seed: a value set by BKIN client software to seed the pseudorandom number generator. This value must be changed from the default whenever a task is loaded or reset to allow the control stateflow to randomize blocks.
      |
      | use_task_protocol_block_sequence_flag: a flag set by the block mask indicating whether to use the task protocol's block sequence (1) or to use a block sequence specified by the task program (0). In the latter case, the block will be given a new
      | input to which a user can input the block table row defining the block that should be run next. This input will be checked when a block (including any repeat trials) is finished in response to the end trial event.
      |
      | next_task_program_specified_block: a value specifying the index of the next block to run if the use_task_protocol_block_sequence_flag is not set. When that flag is not set and a block (including any repeated trials) is finished in response to the
      | end trial event, this input will be used to select the next block to run.
  repeat_trial_flag : Inport
  e_End_Trial : Inport  Port=2
  use_repeat_trial_flag : Inport  Port=3
  run_command : Inport  Port=4
  pause_type : Inport  Port=5
  seed : Inport  Port=6
  use_task_protocol_block_sequence_flag : Inport  Port=7
  next_task_program_specified_block : Inport  Port=8
  run_task_clock_flag : Inport  Port=9
  Compare To Constant : simulink/Logic and Bit Operations/Compare To Constant  relop===  const=2.0  OutDataTypeStr=uint8  ZeroCross=off
  Constant : Constant
  Data Type Conversion : DataTypeConversion
  Data Type Conversion1 : DataTypeConversion
  Data Type Conversion2 : DataTypeConversion  OutDataTypeStr=double
  Delay : Memory
  Delay1 : Memory
  Mux1 : Mux  Inputs=2
  Mux2 : Mux  Inputs=2
  Product : Product  RndMeth=Zero
  Product2 : Product  RndMeth=Zero
  Product3 : Product  RndMeth=Zero
  Selector : Selector  NumberOfDimensions=2  InputPortWidth=3  IndexOptions=Select all,Index vector (dialog)  Indices=-1,1  OutputSizes=slselsubs([(-2),(-2)],1),slselsubs([(-2),(-2)],2)
  Selector1 : Selector  NumberOfDimensions=2  InputPortWidth=3  IndexOptions=Index vector (dialog),Select all  Indices=1,-1  OutputSizes=slselsubs([(-2),(-2)],1),slselsubs([(-2),(-2)],2)
  Selector2 : Selector  NumberOfDimensions=2  InputPortWidth=3  IndexOptions=Select all,Index vector (dialog)  Indices=-1,1  OutputSizes=slselsubs([(-2),(-2)],1),slselsubs([(-2),(-2)],2)
  Subtract : Sum  Inputs=+-  OutDataTypeStr=Inherit: Inherit via back propagation
  Task Clock : DiscretePulseGenerator  PulseType=Time based  Period=.001  PulseWidth=50  SampleTime=0.0005
  Task Execution Control Machine : Stateflow chart  TreatAsAtomicUnit=on
  Width : Width  DataType=uint32
  Width1 : Width  DataType=uint32
  Width2 : Width  DataType=uint32
  trial_control : Outport
  tp : Outport  Port=2
  block : Outport  Port=3
  trial_in_block : Outport  Port=4
  block_in_set : Outport  Port=5
  trial_in_set : Outport  Port=6
  global_clock : Outport  Port=7
  run_status : Outport  Port=8
  run_state : Outport  Port=9
  wires:
  Data Type Conversion2/1 -> run_status/1
  Task Clock/1 -> Product/2
  run_task_clock_flag/1 -> Product/1
  Width2/1 -> Task Execution Control Machine/10(task_protocol_block_sequence_length)
  Selector2/1 -> Width2/1
  Width1/1 -> Subtract/1
  Subtract/1 -> Task Execution Control Machine/7(trial_queue_max_length)
  Selector1/1 -> Width1/1
  Constant/1 -> Subtract/2
  Selector/1 -> Width/1
  Width/1 -> Task Execution Control Machine/6(max_block_definitions)
  [Block_Sequence] -> Selector2/1, Task Execution Control Machine/9(task_protocol_block_sequence)
  use_task_protocol_block_sequence_flag/1 -> Task Execution Control Machine/8(use_task_protocol_block_sequence_flag)
  [Block_Definitions] -> Selector1/1, Selector/1, Task Execution Control Machine/5(block_definitions)
  Data Type Conversion1/1 -> Mux2/1
  Product2/1 -> Data Type Conversion1/1
  Compare To Constant/1 -> Data Type Conversion2/1, Product2/2
  next_task_program_specified_block/1 -> Task Execution Control Machine/11(next_task_program_specified_block)
  Task Execution Control Machine/1(task_status) -> run_state/1, Compare To Constant/1
  use_repeat_trial_flag/1 -> Product3/2
  Delay1/1 -> Product3/1
  repeat_trial_flag/1 -> Delay1/1
  Task Execution Control Machine/3(block) -> block/1
  Task Execution Control Machine/4(trial_in_block) -> trial_in_block/1
  Task Execution Control Machine/5(block_in_set) -> block_in_set/1
  Product3/1 -> Task Execution Control Machine/1(repeat_trial_flag)
  Product/1 -> Mux1/1, global_clock/1, Product2/1
  Delay/1 -> Data Type Conversion/1
  Data Type Conversion/1 -> Mux1/2
  Mux1/1 -> Task Execution Control Machine/Trigger
  Task Execution Control Machine/7(e_exit_trial) -> Mux2/2
  Mux2/1 -> trial_control/1
  e_End_Trial/1 -> Delay/1
  run_command/1 -> Task Execution Control Machine/2(run_command)
  pause_type/1 -> Task Execution Control Machine/3(pause_type)
  Task Execution Control Machine/6(trial_in_set) -> trial_in_set/1
  Task Execution Control Machine/2(tp) -> tp/1
  seed/1 -> Task Execution Control Machine/4(seed)

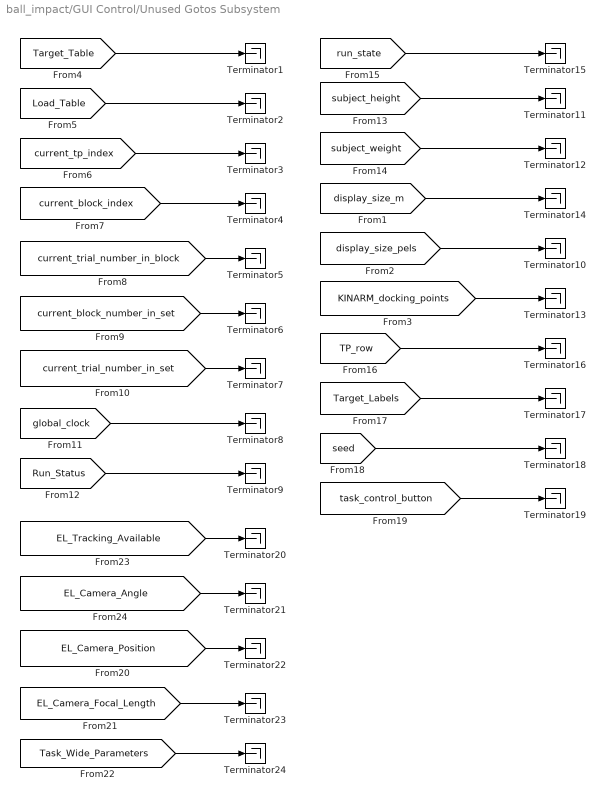
== system ball_impact/GUI Control/Unused Gotos Subsystem ==
  Terminator{1..24} (24 alike) : Terminator
  wires:
  [task_control_button] -> Terminator19/1
  [seed] -> Terminator18/1
  [Target_Labels] -> Terminator17/1
  [TP_row] -> Terminator16/1
  [run_state] -> Terminator15/1
  [KINARM_docking_points] -> Terminator13/1
  [display_size_pels] -> Terminator10/1
  [display_size_m] -> Terminator14/1
  [subject_weight] -> Terminator12/1
  [subject_height] -> Terminator11/1
  [Run_Status] -> Terminator9/1
  [global_clock] -> Terminator8/1
  [current_trial_number_in_set] -> Terminator7/1
  [current_block_number_in_set] -> Terminator6/1
  [Target_Table] -> Terminator1/1
  [current_tp_index] -> Terminator3/1
  [Load_Table] -> Terminator2/1
  [current_trial_number_in_block] -> Terminator5/1
  [current_block_index] -> Terminator4/1
  [Task_Wide_Parameters] -> Terminator24/1
  [EL_Camera_Focal_Length] -> Terminator23/1
  [EL_Camera_Position] -> Terminator22/1
  [EL_Camera_Angle] -> Terminator21/1
  [EL_Tracking_Available] -> Terminator20/1

== system ball_impact/Parameter Table Defn/TP_table ==
  BallTarget;BallTarget;target;Target Table row of the ball graphic (X and Y overridden each tick);;;none;; : Constant  Value=2
  HoldTime;HoldTime;int;Required hold at home before release (ms);;;none;; : Constant  Value=4
  HomeTarget;HomeTarget;target;Target Table row of the home target;;;none;; : Constant
  Load;Load;load;Load Table row for this trial;;;none;; : Constant  Value=3
  ReleaseDelayMax;ReleaseDelayMax;int;Maximum random delay before ball release (ms);;;none;; : Constant  Value=6
  ReleaseDelayMin;ReleaseDelayMin;int;Minimum random delay before ball release (ms);;;none;; : Constant  Value=5
  Terminator{1..7} (7 alike) : Terminator
  TrialTimeout;TrialTimeout;int;Maximum trial duration (ms);;;none;; : Constant  Value=7
  wires:
  HomeTarget;HomeTarget;target;Target Table row of the home target;;;none;;/1 -> Terminator1/1
  BallTarget;BallTarget;target;Target Table row of the ball graphic (X and Y overridden each tick);;;none;;/1 -> Terminator2/1
  Load;Load;load;Load Table row for this trial;;;none;;/1 -> Terminator3/1
  HoldTime;HoldTime;int;Required hold at home before release (ms);;;none;;/1 -> Terminator4/1
  ReleaseDelayMin;ReleaseDelayMin;int;Minimum random delay before ball release (ms);;;none;;/1 -> Terminator5/1
  ReleaseDelayMax;ReleaseDelayMax;int;Maximum random delay before ball release (ms);;;none;;/1 -> Terminator6/1
  TrialTimeout;TrialTimeout;int;Maximum trial duration (ms);;;none;;/1 -> Terminator7/1

== system ball_impact/Parameter Table Defn/buttons ==
  BTN_MARK;Mark event;;Marks a timestamp event in the data;;;;; : Constant  Value=2
  BTN_REPEAT;Repeat trial;;Repeat the current trial;;;;; : Constant  Value=3
  Terminator1 : Terminator
  Terminator2 : Terminator
  wires:
  BTN_MARK;Mark event;;Marks a timestamp event in the data;;;;;/1 -> Terminator1/1
  BTN_REPEAT;Repeat trial;;Repeat the current trial;;;;;/1 -> Terminator2/1
